simulink model "EspacoDeEstadosDiscreto"  (R2026a)
settings: Solver=VariableStepAuto
values from neighbouring files (symbols this model uses):
  Ad = expm(A*Ts)    [paramEmc.m]
  Bd = integral(@(t) expm(A*t)*B,0,Ts,'ArrayValued',true)    [paramEmc.m]
  Cd = C    [paramEmc.m]
  Kd = place(Ad, Bd, polos_desejados_discretos)    [paramEmc.m]
  Ts = 0.001    [paramEmc.m]
  x0 = [deg2rad(12); 0; 0]    [paramEmc.m]
settings Model: Creator=Agmar  LastModifiedBy=Enzo

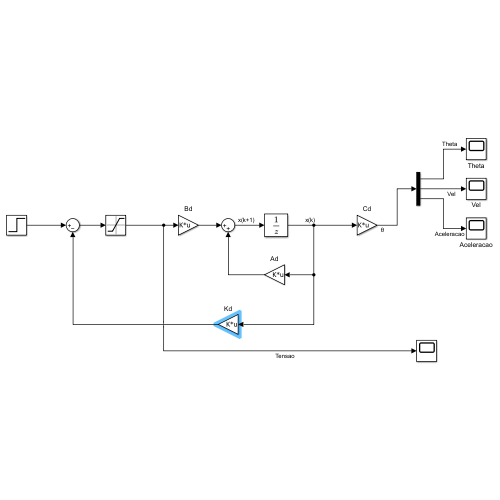
[thumbnail: Simulink's stored preview of the top-level diagram]
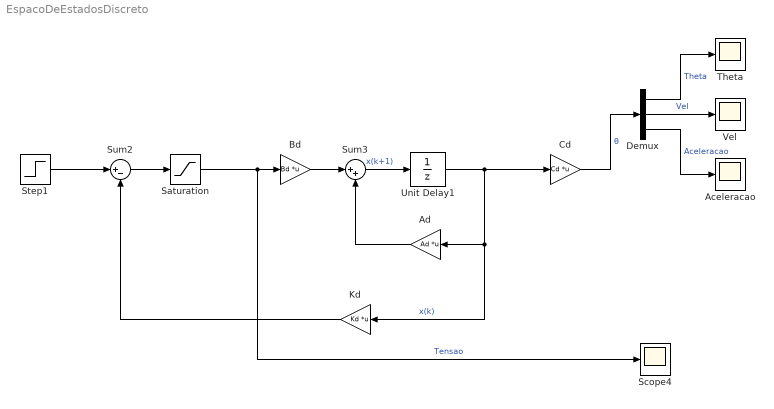
== system EspacoDeEstadosDiscreto ==
  Aceleracao : Scope
      settings: ActiveDisplayYMinimum=-2.773601751689029  ActiveDisplayYMaximum=24.962415765201264
  Ad : Gain  Gain=Ad  Multiplication=Matrix(K*u)
  Bd : Gain  Gain=Bd  Multiplication=Matrix(K*u)
  Cd : Gain  Gain=Cd  Multiplication=Matrix(K*u)
  Demux : Demux  Outputs=3
  Kd : Gain  Gain=Kd  Multiplication=Matrix(K*u)
  Saturation : Saturate  UpperLimit=18  LowerLimit=-18
  Scope4 : Scope
      settings: ActiveDisplayYMinimum=-2.2499999999999996  ActiveDisplayYMaximum=20.25  DataLoggingVariableName=ScopeData4
  Step1 : Step  Time=0  FinalValue=0  SampleTime=0
  Sum2 : Sum  Inputs=|+-
  Sum3 : Sum  Inputs=|++
  Theta : Scope
      settings: ActiveDisplayYMinimum=-0.079242898694786942  ActiveDisplayYMaximum=0.2415153334542203
  Unit Delay1 : UnitDelay  InitialCondition=x0  SampleTime=Ts
  Vel : Scope
      settings: ActiveDisplayYMinimum=-1.8441472359809239  ActiveDisplayYMaximum=0.40453205360899214  DataLoggingVariableName=ScopeData3
  wires:
  Sum2/1 -> Saturation/1
  Saturation/1 -> Scope4/1, Bd/1  "Tensao"
  Step1/1 -> Sum2/1
  Kd/1 -> Sum2/2
  Sum3/1 -> Unit Delay1/1  "x(k+1)"
  Ad/1 -> Sum3/2
  Bd/1 -> Sum3/1
  Unit Delay1/1 -> Kd/1, Ad/1, Cd/1  "x(k)"
  Cd/1 -> Demux/1  "θ"
  Demux/2 -> Vel/1  "Vel"
  Demux/1 -> Theta/1  "Theta"
  Demux/3 -> Aceleracao/1  "Aceleracao"
